simulink library "SCR"  (R2024b)
settings: Solver=VariableStepAuto  StartTime=0.0  StopTime=10.0  RelTol=1e-3
libraries: nesl_utility x29, fl_lib x26, sm_lib x16, ee_lib x7, slpidlib x4
(part 2 of 2)

== system SCR/PID Controller ==
  q1 : Inport
  Q_dorit : Inport  Port=2
  q2 : Inport  Port=3
  Add : Sum  Inputs=-+
  Add1 : Sum  Inputs=+-
  Demux : Demux  Outputs=2
  Mux : Mux  Inputs=2
  Mux1 : Mux  Inputs=2
  PID Controller : slpidlib/PID Controller  Controller=PID  Form=Parallel  TimeDomain=Continuous-time  UseExternalTs=off  SampleTime=-1  IntegratorMethod=Forward Euler  FilterMethod=Forward Euler  ControllerParametersSource=internal  P=17042.9277196606  I=696153.474275857  UseKiTs=off  D=-7.42275649016862  UseExternalDerivativeSource=off  N=2296.03756262702  UseFilter=on  TunerSelectOption=Transfer Function Based (PID Tuner App)  InitialConditionSource=internal  InitialConditionForIntegrator=0  InitialConditionForFilter=0  DifferentiatorICPrevScaledInput=0  ExternalReset=none  TrackingMode=off  Kt=1  LimitOutput=on  SatLimitsSource=internal  UpperSaturationLimit=24  LowerSaturationLimit=-24  LinearizeAsGain=off  AntiWindupMode=clamping  Kb=10  LimitIntegrator=off  UpperIntegratorSaturationLimit=inf  LowerIntegratorSaturationLimit=-inf  POutMin=[]  POutMax=[]  IOutMin=[]  IOutMax=[]  DOutMin=[]  DOutMax=[]  NOutMin=[]  NOutMax=[]  SumOutMin=[]  SumOutMax=[]  SaturationOutMin=[]  SaturationOutMax=[]  PParamMin=[]  PParamMax=[]  IParamMin=[]  IParamMax=[]  DParamMin=[]  DParamMax=[]  NParamMin=[]  NParamMax=[]  KbParamMin=[]  KbParamMax=[]  KtParamMin=[]  KtParamMax=[]  KbOutMin=[]  KbOutMax=[]  KtOutMin=[]  KtOutMax=[]  IntegratorOutMin=[]  IntegratorOutMax=[]  FilterOutMin=[]  FilterOutMax=[]  SumI1OutMin=[]  SumI1OutMax=[]  SumI2OutMin=[]  SumI2OutMax=[]  SumI3OutMin=[]  SumI3OutMax=[]  SumI4OutMin=[]  SumI4OutMax=[]  SumDOutMin=[]  SumDOutMax=[]  DifferentiatorOutMin=[]  DifferentiatorOutMax=[]  FilterDiffOutCoefMin=[]  FilterDiffOutCoefMax=[]  ReciprocalOutMin=[]  ReciprocalOutMax=[]  SumDenOutMin=[]  SumDenOutMax=[]  SumNumOutMin=[]  SumNumOutMax=[]  DivideOutMin=[]  DivideOutMax=[]  UdiffTsProdOutMin=[]  UdiffTsProdOutMax=[]  NTsProdOutMin=[]  NTsProdOutMax=[]  UintegralTsProdOutMin=[]  UintegralTsProdOutMax=[]  UngainTsProdOutMin=[]  UngainTsProdOutMax=[]  ClampingZeroOutDataTypeStr=Inherit: Inherit via back propagation  ClampingZeroOutMin=[]  ClampingZeroOutMax=[]  FilterDenConstantOutDataTypeStr=Inherit: Inherit via back propagation  FilterDenConstantOutMin=[]  FilterDenConstantOutMax=[]  PCopyOutDataTypeStr=Inherit: Inherit via back propagation  PCopyOutMin=[]  PCopyOutMax=[]  NCopyOutDataTypeStr=Inherit: Inherit via back propagation  NCopyOutMin=[]  NCopyOutMax=[]  IntegratorContinuousStateAttributes=''  IntegratorStateMustResolveToSignalObject=off  IntegratorRTWStateStorageClass=Auto  FilterContinuousStateAttributes=''  FilterStateMustResolveToSignalObject=off  FilterRTWStateStorageClass=Auto  ParallelPVariant=InternalParameters  IdealPVariant=Disabled  IVariant=InternalParameters  DVariant=InternalParameters  IntegratorVariant=Continuous  SatVariant=Enabled  AWVariant=ContClampingParallel  PCopyVariant=Disabled  TRVariant=Disabled  FdbkBlocksVariant=Forward  IdealPFdbkVariant=Disabled  SatFdbkVariant=Disabled  DerivativeFilterVariant=ContFilter  NVariant=InternalParameters  NCopyVariant=Disabled  FilterICVariant=InternalICsFilter  IntegratorICVariant=InternalICs  ExternalResetVariant=Disabled  TRSumVariant=Passthrough  SumFdbkVariant=Disabled  SumVariant=Sum_PID  TsampFilterVariant=InternalTs  TsampNgainVariant=Passthrough  TsampIntegralVariant=Disabled_SignalSpec  ExternalSaturationOutDataTypeStr=Inherit: Same as second input  DerivativeSourceVariant=ErrorSignal  PreIntVariant=InternalPreInt
  PID Controller2 : slpidlib/PID Controller  Controller=PID  Form=Parallel  TimeDomain=Continuous-time  UseExternalTs=off  SampleTime=-1  IntegratorMethod=Forward Euler  FilterMethod=Forward Euler  ControllerParametersSource=internal  P=19726.0931917022  I=877163.671153983  UseKiTs=off  D=28.399075244163  UseExternalDerivativeSource=off  N=2735.67202823723  UseFilter=on  TunerSelectOption=Transfer Function Based (PID Tuner App)  InitialConditionSource=internal  InitialConditionForIntegrator=0  InitialConditionForFilter=0  DifferentiatorICPrevScaledInput=0  ExternalReset=none  TrackingMode=off  Kt=1  LimitOutput=on  SatLimitsSource=internal  UpperSaturationLimit=24  LowerSaturationLimit=-24  LinearizeAsGain=off  AntiWindupMode=clamping  Kb=10  LimitIntegrator=off  UpperIntegratorSaturationLimit=inf  LowerIntegratorSaturationLimit=-inf  POutMin=[]  POutMax=[]  IOutMin=[]  IOutMax=[]  DOutMin=[]  DOutMax=[]  NOutMin=[]  NOutMax=[]  SumOutMin=[]  SumOutMax=[]  SaturationOutMin=[]  SaturationOutMax=[]  PParamMin=[]  PParamMax=[]  IParamMin=[]  IParamMax=[]  DParamMin=[]  DParamMax=[]  NParamMin=[]  NParamMax=[]  KbParamMin=[]  KbParamMax=[]  KtParamMin=[]  KtParamMax=[]  KbOutMin=[]  KbOutMax=[]  KtOutMin=[]  KtOutMax=[]  IntegratorOutMin=[]  IntegratorOutMax=[]  FilterOutMin=[]  FilterOutMax=[]  SumI1OutMin=[]  SumI1OutMax=[]  SumI2OutMin=[]  SumI2OutMax=[]  SumI3OutMin=[]  SumI3OutMax=[]  SumI4OutMin=[]  SumI4OutMax=[]  SumDOutMin=[]  SumDOutMax=[]  DifferentiatorOutMin=[]  DifferentiatorOutMax=[]  FilterDiffOutCoefMin=[]  FilterDiffOutCoefMax=[]  ReciprocalOutMin=[]  ReciprocalOutMax=[]  SumDenOutMin=[]  SumDenOutMax=[]  SumNumOutMin=[]  SumNumOutMax=[]  DivideOutMin=[]  DivideOutMax=[]  UdiffTsProdOutMin=[]  UdiffTsProdOutMax=[]  NTsProdOutMin=[]  NTsProdOutMax=[]  UintegralTsProdOutMin=[]  UintegralTsProdOutMax=[]  UngainTsProdOutMin=[]  UngainTsProdOutMax=[]  ClampingZeroOutDataTypeStr=Inherit: Inherit via back propagation  ClampingZeroOutMin=[]  ClampingZeroOutMax=[]  FilterDenConstantOutDataTypeStr=Inherit: Inherit via back propagation  FilterDenConstantOutMin=[]  FilterDenConstantOutMax=[]  PCopyOutDataTypeStr=Inherit: Inherit via back propagation  PCopyOutMin=[]  PCopyOutMax=[]  NCopyOutDataTypeStr=Inherit: Inherit via back propagation  NCopyOutMin=[]  NCopyOutMax=[]  IntegratorContinuousStateAttributes=''  IntegratorStateMustResolveToSignalObject=off  IntegratorRTWStateStorageClass=Auto  FilterContinuousStateAttributes=''  FilterStateMustResolveToSignalObject=off  FilterRTWStateStorageClass=Auto  ParallelPVariant=InternalParameters  IdealPVariant=Disabled  IVariant=InternalParameters  DVariant=InternalParameters  IntegratorVariant=Continuous  SatVariant=Enabled  AWVariant=ContClampingParallel  PCopyVariant=Disabled  TRVariant=Disabled  FdbkBlocksVariant=Forward  IdealPFdbkVariant=Disabled  SatFdbkVariant=Disabled  DerivativeFilterVariant=ContFilter  NVariant=InternalParameters  NCopyVariant=Disabled  FilterICVariant=InternalICsFilter  IntegratorICVariant=InternalICs  ExternalResetVariant=Disabled  TRSumVariant=Passthrough  SumFdbkVariant=Disabled  SumVariant=Sum_PID  TsampFilterVariant=InternalTs  TsampNgainVariant=Passthrough  TsampIntegralVariant=Disabled_SignalSpec  ExternalSaturationOutDataTypeStr=Inherit: Same as second input  DerivativeSourceVariant=ErrorSignal  PreIntVariant=InternalPreInt
  To Workspace : ToWorkspace  VariableName=comanda  SaveFormat=Timeseries  SampleTime=-1
  To Workspace1 : ToWorkspace  VariableName=erori_Q  SaveFormat=Timeseries  SampleTime=-1
  u1 : Outport
  u2 : Outport  Port=2
  wires:
  Demux/2 -> Add1/1
  Demux/1 -> Add/2
  q1/1 -> Add/1
  Add/1 -> Mux1/1, PID Controller/1
  Q_dorit/1 -> Demux/1
  Add1/1 -> PID Controller2/1, Mux1/2
  q2/1 -> Add1/2
  PID Controller/1 -> Mux/1, u1/1  "u1"
  PID Controller2/1 -> Mux/2, u2/1  "u2"
  Mux/1 -> To Workspace/1
  Mux1/1 -> To Workspace1/1

== system SCR/Q_sensed ==
  q1 : Inport
  q2 : Inport  Port=2
  Mux : Mux  Inputs=2
  q_sensor : Outport
  tag scope: q1=global, q2=global, q_sensor=global
  wires:
  q1/1 -> Mux/1, [q1]
  q2/1 -> Mux/2, [q2]
  Mux/1 -> q_sensor/1, [q_sensor]

== system SCR/SCARA_FD_Holist ==
  u : Inport
  Demux : Demux  Outputs=2
  Demux1 : Demux  Outputs=2
  Demux2 : Demux  Outputs=2
  Integrator : Integrator
  Integrator1 : Integrator
  ddq compute : MATLAB Function  TreatAsAtomicUnit=on
  q1 : Outport
  q2 : Outport  Port=2
  dq1 : Outport  Port=3
  dq2 : Outport  Port=4
  ddq1 : Outport  Port=5
  ddq2 : Outport  Port=6
  wires:
  Demux2/2 -> q2/1, ddq compute/2(q2)
  Demux2/1 -> q1/1
  Integrator1/1 -> Demux2/1
  Demux1/2 -> dq2/1, ddq compute/4(dq2)
  Demux1/1 -> dq1/1, ddq compute/3(dq1)
  Demux/2 -> ddq2/1
  Demux/1 -> ddq1/1
  Integrator/1 -> Integrator1/1, Demux1/1
  u/1 -> ddq compute/1(u)
  ddq compute/1(ddq) -> Demux/1, Integrator/1

== system SCR/SCARA_Foward_Dynamics ==
  tau : Inport
  Demux : Demux  Outputs=2
  Demux1 : Demux  Outputs=2
  Demux2 : Demux  Outputs=2
  Integrator : Integrator
  Integrator1 : Integrator
  ddq compute : MATLAB Function  TreatAsAtomicUnit=on
  q1 : Outport
  q2 : Outport  Port=2
  dq1 : Outport  Port=3
  dq2 : Outport  Port=4
  ddq1 : Outport  Port=5
  ddq2 : Outport  Port=6
  wires:
  ddq compute/1(ddq) -> Integrator/1, Demux/1
  tau/1 -> ddq compute/1(tau)
  Integrator/1 -> Demux1/1, Integrator1/1
  Demux/1 -> ddq1/1
  Demux/2 -> ddq2/1
  Demux1/1 -> ddq compute/3(dq1), dq1/1
  Demux1/2 -> ddq compute/4(dq2), dq2/1
  Integrator1/1 -> Demux2/1
  Demux2/1 -> q1/1
  Demux2/2 -> ddq compute/2(q2), q2/1

== system SCR/SCARA_Inverse_Dynamics ==
  q,dq,ddq : Inport
  Demux : Demux  Outputs=2
  Demux1 : Demux  Outputs=5
  Memory : Memory
  To Workspace : ToWorkspace  VariableName=torque  SaveFormat=Timeseries  SampleTime=-1
  tau compute : MATLAB Function  TreatAsAtomicUnit=on
  Torque Joint1 : Outport
  Torque Joint2 : Outport  Port=2
  wires:
  Memory/1 -> Demux1/1
  Demux1/5 -> tau compute/5(ddq2)
  Demux1/4 -> tau compute/4(dq2)
  Demux1/3 -> tau compute/3(q2)
  Demux1/2 -> tau compute/2(ddq1)
  Demux1/1 -> tau compute/1(dq1)
  q,dq,ddq/1 -> Memory/1
  Demux/1 -> Torque Joint1/1
  Demux/2 -> Torque Joint2/1
  tau compute/1(tau) -> To Workspace/1, Demux/1

== system SCR/Scope current, voltage, RPM ==
  Scope : Scope  NumInputPorts=2
  Scope1 : Scope  NumInputPorts=2
  Scope2 : Scope  NumInputPorts=2
  wires:
  [motorCurrent1] -> Scope/1
  [motorCurrent2] -> Scope/2
  [motorVoltage2] -> Scope1/2
  [motorVoltage1] -> Scope1/1
  [motorRPM1] -> Scope2/1
  [motorRPM2] -> Scope2/2

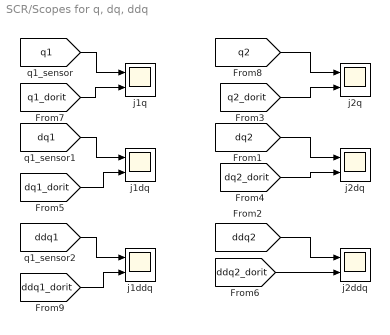
== system SCR/Scopes for q, dq, ddq ==
  j1ddq : Scope  NumInputPorts=2
  j1dq : Scope  NumInputPorts=2
  j1q : Scope  NumInputPorts=2
  j2ddq : Scope  NumInputPorts=2
  j2dq : Scope  NumInputPorts=2
  j2q : Scope  NumInputPorts=2
  wires:
  [dq1] -> j1dq/1
  [q2] -> j2q/1
  [q1] -> j1q/1
  [ddq2] -> j2ddq/1
  [ddq1] -> j1ddq/1
  [dq2] -> j2dq/1
  [dq1_dorit] -> j1dq/2
  [q1_dorit] -> j1q/2
  [ddq1_dorit] -> j1ddq/2
  [q2_dorit] -> j2q/2
  [ddq2_dorit] -> j2ddq/2
  [dq2_dorit] -> j2dq/2

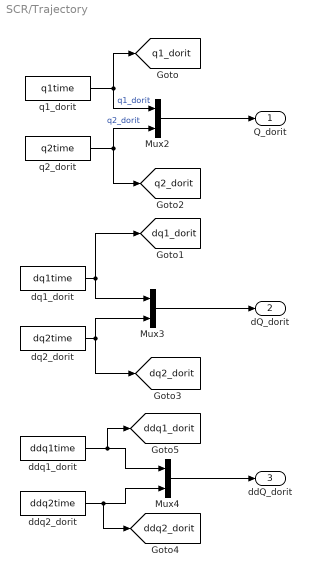
== system SCR/Trajectory ==
  Mux2 : Mux  Inputs=2
  Mux3 : Mux  Inputs=2
  Mux4 : Mux  Inputs=2
  ddq1_dorit : FromWorkspace  VariableName=ddq1time
  ddq2_dorit : FromWorkspace  VariableName=ddq2time
  dq1_dorit : FromWorkspace  VariableName=dq1time
  dq2_dorit : FromWorkspace  VariableName=dq2time
  q1_dorit : FromWorkspace  VariableName=q1time
  q2_dorit : FromWorkspace  VariableName=q2time
  Q_dorit : Outport
  dQ_dorit : Outport  Port=2
  ddQ_dorit : Outport  Port=3
  tag scope: ddq1_dorit=global, ddq2_dorit=global, dq1_dorit=global, dq2_dorit=global, q1_dorit=global, q2_dorit=global
  wires:
  Mux4/1 -> ddQ_dorit/1
  Mux2/1 -> Q_dorit/1
  Mux3/1 -> dQ_dorit/1
  q2_dorit/1 -> Mux2/2, [q2_dorit]  "q2_dorit"
  q1_dorit/1 -> Mux2/1, [q1_dorit]  "q1_dorit"
  dq1_dorit/1 -> [dq1_dorit], Mux3/1
  dq2_dorit/1 -> Mux3/2, [dq2_dorit]
  ddq1_dorit/1 -> [ddq1_dorit], Mux4/1
  ddq2_dorit/1 -> [ddq2_dorit], Mux4/2

== system SCR/actuatorTorques ==
  Actuator Torque 1 : Inport
  Actuator Torque 2 : Inport  Port=2
  Mux : Mux  Inputs=2
  tag scope: actuatorTorque1=global, actuatorTorque2=global, actuatorTorques=global
  wires:
  Actuator Torque 1/1 -> Mux/1, [actuatorTorque1]
  Actuator Torque 2/1 -> Mux/2, [actuatorTorque2]
  Mux/1 -> [actuatorTorques]

== system SCR/dQ_sensed ==
  dq1 : Inport
  dq2 : Inport  Port=2
  Mux1 : Mux  Inputs=2
  dq_sensor : Outport
  tag scope: dq1=global, dq2=global, dq_sensor=global
  wires:
  dq1/1 -> [dq1], Mux1/1
  dq2/1 -> Mux1/2, [dq2]
  Mux1/1 -> dq_sensor/1, [dq_sensor]

== system SCR/ddQ_sensed ==
  ddq1 : Inport
  ddq2 : Inport  Port=2
  Mux1 : Mux  Inputs=2
  tag scope: ddq1=global, ddq2=global, ddq_sensor=global
  wires:
  ddq1/1 -> [ddq1], Mux1/1
  ddq2/1 -> [ddq2], Mux1/2
  Mux1/1 -> [ddq_sensor]

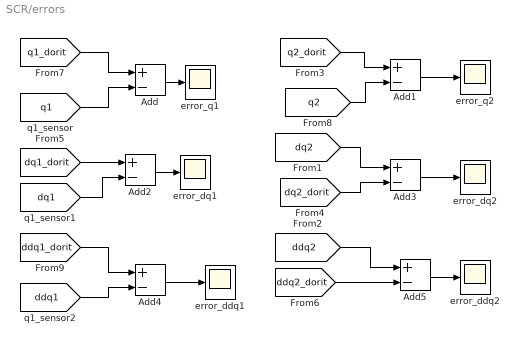
== system SCR/errors ==
  Add{,1..5} (6 alike) : Sum  Inputs=+-
  error_ddq1 : Scope
  error_ddq2 : Scope
  error_dq1 : Scope
  error_dq2 : Scope
  error_q1 : Scope
  error_q2 : Scope
  wires:
  [ddq2] -> Add5/1
  [ddq2_dorit] -> Add5/2
  Add/1 -> error_q1/1
  [q1_dorit] -> Add/1
  [q1] -> Add/2
  [q2_dorit] -> Add1/1
  [q2] -> Add1/2
  Add1/1 -> error_q2/1
  [dq1_dorit] -> Add2/1
  Add2/1 -> error_dq1/1
  [dq1] -> Add2/2
  Add3/1 -> error_dq2/1
  [dq2] -> Add3/1
  [dq2_dorit] -> Add3/2
  [ddq1_dorit] -> Add4/1
  [ddq1] -> Add4/2
  Add4/1 -> error_ddq1/1
  Add5/1 -> error_ddq2/1

== system SCR/Controller_ID/Subsystem ==
  q1 : Inport
  q2 : Inport  Port=2
  dq1 : Inport  Port=3
  dq2 : Inport  Port=4
  MATLAB Function1 : MATLAB Function  TreatAsAtomicUnit=on
  MATLAB Function2 : MATLAB Function  TreatAsAtomicUnit=on
  MATLAB Function3 : MATLAB Function  TreatAsAtomicUnit=on
  M : Outport
  N : Outport  Port=2
  G : Outport  Port=3
  wires:
  MATLAB Function3/1(M) -> M/1
  MATLAB Function1/1(N) -> N/1
  q2/1 -> MATLAB Function2/2(q2), MATLAB Function1/1(q2), MATLAB Function3/1(q2)
  dq2/1 -> MATLAB Function1/3(dq2)
  dq1/1 -> MATLAB Function1/2(dq1)
  MATLAB Function2/1(G) -> G/1
  q1/1 -> MATLAB Function2/1(q1)

== system SCR/Feedfoward/Subsystem ==
  q1 : Inport
  q2 : Inport  Port=2
  dq1 : Inport  Port=3
  dq2 : Inport  Port=4
  MATLAB Function1 : MATLAB Function  TreatAsAtomicUnit=on
  MATLAB Function2 : MATLAB Function  TreatAsAtomicUnit=on
  MATLAB Function3 : MATLAB Function  TreatAsAtomicUnit=on
  M : Outport
  N : Outport  Port=2
  G : Outport  Port=3
  wires:
  MATLAB Function3/1(M) -> M/1
  MATLAB Function1/1(N) -> N/1
  q2/1 -> MATLAB Function2/2(q2), MATLAB Function1/1(q2), MATLAB Function3/1(q2)
  dq2/1 -> MATLAB Function1/3(dq2)
  dq1/1 -> MATLAB Function1/2(dq1)
  MATLAB Function2/1(G) -> G/1
  q1/1 -> MATLAB Function2/1(q1)

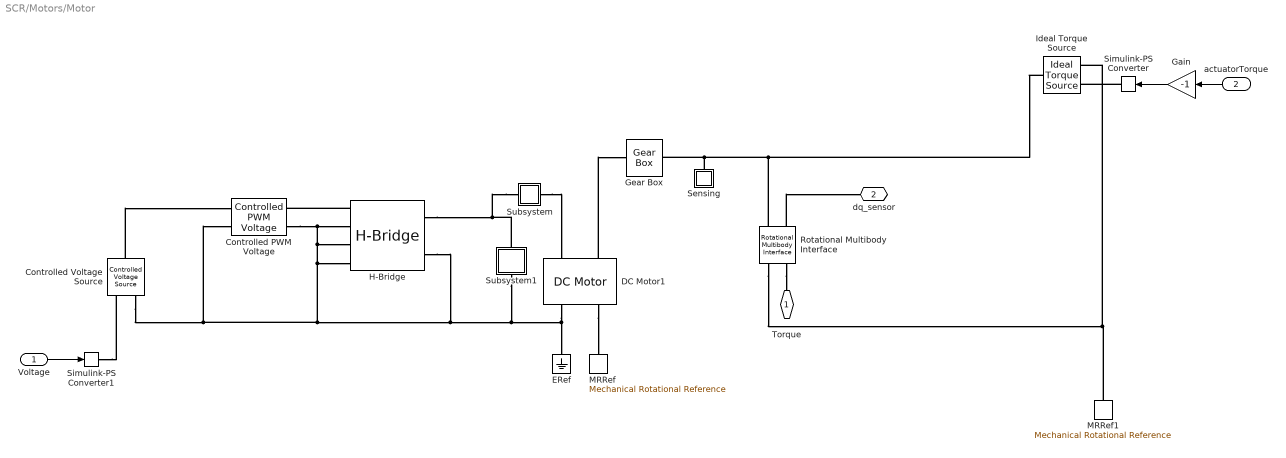
== system SCR/Motors/Motor ==
  Voltage : Inport
  actuatorTorque : Inport  Port=2
  Controlled PWM Voltage : ee_lib/Integrated Circuits/Controlled PWM Voltage  F=4000 Hz  TD=0 s  pulse_width_offset=0 s  pulse_min=0 s  pwm_or_av=ee.enum.pwm_or_av.averaged  event_type=1  sample_time=5e-6 s  Vmin=0 V  Vmax=5 V  Vm=5 V  u_min=0  u_max=1
  Controlled Voltage Source : fl_lib/Electrical/Electrical Sources/Controlled Voltage Source
  DC Motor1 : ee_lib/Electromechanical/Brushed Motors/DC Motor  field_option=ee.enum.field_option.pm  Rf=100 Ohm  Lf=1 H  Laf=0.15 H  If0=0 A  parameterization=ee.enum.dcparam_option.circuit_param  Ra=3.9 Ohm  La=12e-6 H  emf_or_torque=ee.enum.emf_or_torque.kv  Kv=0.072e-3 V/rpm  Ki=6.876e-4 N*m/A  T_stall=0.24e-3 N*m  w_max=19100 rpm  w_rated=15000 rpm  P_rated=0.08 W  V_rated=1.5 V  lam_param=ee.enum.lam_param.damping  i_noload=0 A  V_i_noload=1.5 V  J=0.01 cm^2*g  lam=0 N*m*s/rad  speed0=0 rpm  t_fault_armature=1 s  t_fault_field=1 s  fault_action=simscape.enum.assert.action.none  alpha=3.93e-3 1/K  Tmeas=25 degC  thermal_mass=100 J/K  initial_temperature=25 degC
  ERef : fl_lib/Electrical/Electrical Elements/Electrical Reference
  Gain : Gain  Gain=-1
  Gear Box : fl_lib/Mechanical/Mechanisms/Gear Box  ratio=103  t_in_specify=off  t_in_priority=None  t_in=0 N*m  t_in_nominal_specify=off  t_in_nominal_value=1  t_in_nominal_unit=N*m  t_out_specify=off  t_out_priority=None  t_out=0 N*m  t_out_nominal_specify=off  t_out_nominal_value=1  t_out_nominal_unit=N*m
  H-Bridge : ee_lib/Semiconductors & Converters/Converters/H-Bridge  supply_ports=ee.enum.supply_ports.hidesupply  pwm_or_av=2  regenerative_braking_mode=2  discontinuous=0  freewheeling_mode=1  Rload=3.38+0.1 Ohm  Lload=1e-5 H  F=4 kHz  Venable=2.5 V  Vmax=5 V  Vreverse=2.5 V  Vbrake=2.5 V  Vm=12 V  Ron=0.1 Ohm  Don=0.1 Ohm  Goff=1e-6 S  Tmeas=298.15 K  Ron2=0.1 Ohm  Don2=0.05 Ohm  Tmeas2=398.15 K  thermal_mass=100 J/K  initial_temperature=298.15 K
  Ideal Torque Source : fl_lib/Mechanical/Mechanical Sources/Ideal Torque Source
  MRRef : fl_lib/Mechanical/Rotational Elements/Mechanical Rotational Reference
  MRRef1 : fl_lib/Mechanical/Rotational Elements/Mechanical Rotational Reference
  Rotational Multibody Interface : fl_lib/Mechanical/Multibody Interfaces/Rotational Multibody Interface
  Sensing : Subsystem
      mask Display: disp('w');
  Simulink-PS Converter : nesl_utility/Simulink-PS Converter  PhysicalDomain=network_engine_domain  SubClassName=ps_input  LeftPortType=input  RightPortType=output  PseudoPeriodic=off  Frequencies=[]  NoiseDistribution=none  NoiseParameters=[]  Unit=1  AffineConversion=off  FilteringAndDerivatives=provide  SimscapeFilterOrder=1  InputFilterTimeConstant=0.001  UdotUserProvided=0
  Simulink-PS Converter1 : nesl_utility/Simulink-PS Converter  PhysicalDomain=network_engine_domain  SubClassName=ps_input  LeftPortType=input  RightPortType=output  PseudoPeriodic=off  Frequencies=[]  NoiseDistribution=none  NoiseParameters=[]  Unit=1  AffineConversion=off  FilteringAndDerivatives=provide  SimscapeFilterOrder=1  InputFilterTimeConstant=0.001  UdotUserProvided=0
  Subsystem : Subsystem
      mask Display: disp("A")
  Subsystem1 : Subsystem
      mask Display: disp("V")
  Torque : PMIOPort  Side=Left
  dq_sensor : PMIOPort  Port=2  Side=Right
  wires:
  Voltage/1 -> Simulink-PS Converter1/1
  Gain/1 -> Simulink-PS Converter/1
  actuatorTorque/1 -> Gain/1
  connections:
  Subsystem/RConn1 -- DC Motor1/LConn1
  Simulink-PS Converter1/RConn1 -- Controlled Voltage Source/RConn1
  Simulink-PS Converter/RConn1 -- Ideal Torque Source/RConn1
  Ideal Torque Source/RConn2 -- MRRef1/LConn1 -- Rotational Multibody Interface/LConn2
  Rotational Multibody Interface/LConn1 -- Torque/RConn1
  Rotational Multibody Interface/RConn1 -- dq_sensor/RConn1
  Controlled Voltage Source/LConn1 -- Controlled PWM Voltage/LConn1
  Subsystem/LConn1 -- Subsystem1/LConn1 -- H-Bridge/RConn1
  Subsystem1/RConn1 -- H-Bridge/RConn2 -- Controlled PWM Voltage/RConn2 -- H-Bridge/LConn2 -- H-Bridge/LConn3 -- H-Bridge/LConn4 -- Controlled PWM Voltage/LConn2 -- Controlled Voltage Source/RConn2 -- DC Motor1/RConn1 -- ERef/LConn1
  Ideal Torque Source/LConn1 -- Rotational Multibody Interface/RConn2 -- Sensing/LConn1 -- Gear Box/RConn1
  DC Motor1/RConn2 -- MRRef/LConn1
  H-Bridge/LConn1 -- Controlled PWM Voltage/RConn1
  DC Motor1/LConn2 -- Gear Box/LConn1

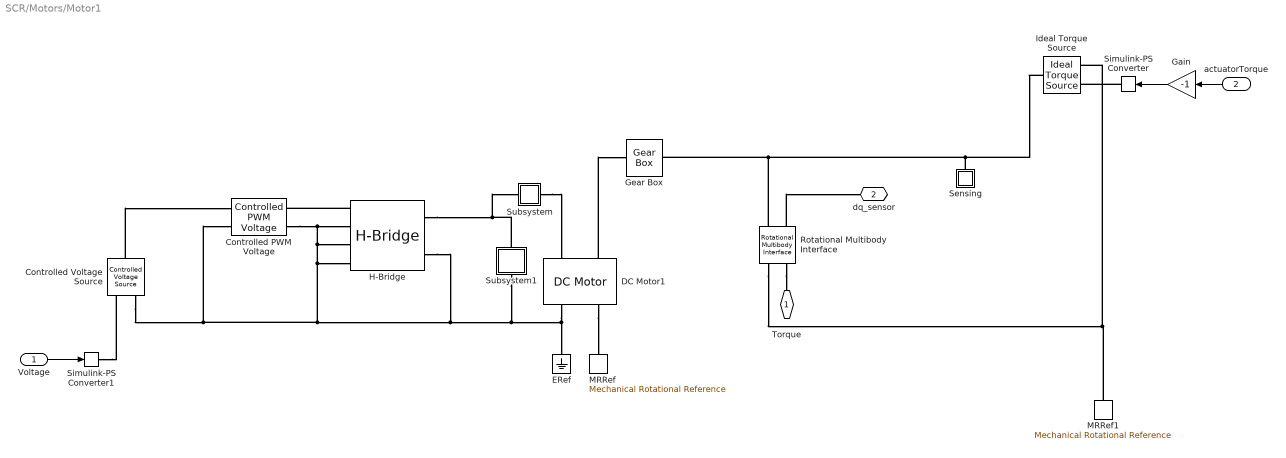
== system SCR/Motors/Motor1 ==
  Voltage : Inport
  actuatorTorque : Inport  Port=2
  Controlled PWM Voltage : ee_lib/Integrated Circuits/Controlled PWM Voltage  F=4000 Hz  TD=0 s  pulse_width_offset=0 s  pulse_min=0 s  pwm_or_av=ee.enum.pwm_or_av.averaged  event_type=1  sample_time=5e-6 s  Vmin=0 V  Vmax=5 V  Vm=5 V  u_min=0  u_max=1
  Controlled Voltage Source : fl_lib/Electrical/Electrical Sources/Controlled Voltage Source
  DC Motor1 : ee_lib/Electromechanical/Brushed Motors/DC Motor  field_option=ee.enum.field_option.pm  Rf=100 Ohm  Lf=1 H  Laf=0.15 H  If0=0 A  parameterization=ee.enum.dcparam_option.circuit_param  Ra=3.9 Ohm  La=12e-6 H  emf_or_torque=ee.enum.emf_or_torque.kv  Kv=0.072e-3 V/rpm  Ki=6.876e-4 N*m/A  T_stall=0.24e-3 N*m  w_max=19100 rpm  w_rated=15000 rpm  P_rated=0.08 W  V_rated=1.5 V  lam_param=ee.enum.lam_param.damping  i_noload=0 A  V_i_noload=1.5 V  J=0.01 cm^2*g  lam=0 N*m*s/rad  speed0=0 rpm  t_fault_armature=1 s  t_fault_field=1 s  fault_action=simscape.enum.assert.action.none  alpha=3.93e-3 1/K  Tmeas=25 degC  thermal_mass=100 J/K  initial_temperature=25 degC
  ERef : fl_lib/Electrical/Electrical Elements/Electrical Reference
  Gain : Gain  Gain=-1
  Gear Box : fl_lib/Mechanical/Mechanisms/Gear Box  ratio=103  t_in_specify=off  t_in_priority=None  t_in=0 N*m  t_in_nominal_specify=off  t_in_nominal_value=1  t_in_nominal_unit=N*m  t_out_specify=off  t_out_priority=None  t_out=0 N*m  t_out_nominal_specify=off  t_out_nominal_value=1  t_out_nominal_unit=N*m
  H-Bridge : ee_lib/Semiconductors & Converters/Converters/H-Bridge  supply_ports=ee.enum.supply_ports.hidesupply  pwm_or_av=2  regenerative_braking_mode=2  discontinuous=0  freewheeling_mode=1  Rload=3.38+0.1 Ohm  Lload=1e-5 H  F=4 kHz  Venable=2.5 V  Vmax=5 V  Vreverse=2.5 V  Vbrake=2.5 V  Vm=12 V  Ron=0.1 Ohm  Don=0.1 Ohm  Goff=1e-6 S  Tmeas=298.15 K  Ron2=0.1 Ohm  Don2=0.05 Ohm  Tmeas2=398.15 K  thermal_mass=100 J/K  initial_temperature=298.15 K
  Ideal Torque Source : fl_lib/Mechanical/Mechanical Sources/Ideal Torque Source
  MRRef : fl_lib/Mechanical/Rotational Elements/Mechanical Rotational Reference
  MRRef1 : fl_lib/Mechanical/Rotational Elements/Mechanical Rotational Reference
  Rotational Multibody Interface : fl_lib/Mechanical/Multibody Interfaces/Rotational Multibody Interface
  Sensing : Subsystem
      mask Display: disp('w');
  Simulink-PS Converter : nesl_utility/Simulink-PS Converter  PhysicalDomain=network_engine_domain  SubClassName=ps_input  LeftPortType=input  RightPortType=output  PseudoPeriodic=off  Frequencies=[]  NoiseDistribution=none  NoiseParameters=[]  Unit=1  AffineConversion=off  FilteringAndDerivatives=provide  SimscapeFilterOrder=1  InputFilterTimeConstant=0.001  UdotUserProvided=0
  Simulink-PS Converter1 : nesl_utility/Simulink-PS Converter  PhysicalDomain=network_engine_domain  SubClassName=ps_input  LeftPortType=input  RightPortType=output  PseudoPeriodic=off  Frequencies=[]  NoiseDistribution=none  NoiseParameters=[]  Unit=1  AffineConversion=off  FilteringAndDerivatives=provide  SimscapeFilterOrder=1  InputFilterTimeConstant=0.001  UdotUserProvided=0
  Subsystem : Subsystem
      mask Display: disp("A")
  Subsystem1 : Subsystem
      mask Display: disp("V")
  Torque : PMIOPort  Side=Left
  dq_sensor : PMIOPort  Port=2  Side=Right
  wires:
  Voltage/1 -> Simulink-PS Converter1/1
  Gain/1 -> Simulink-PS Converter/1
  actuatorTorque/1 -> Gain/1
  connections:
  Subsystem/RConn1 -- DC Motor1/LConn1
  Simulink-PS Converter1/RConn1 -- Controlled Voltage Source/RConn1
  Simulink-PS Converter/RConn1 -- Ideal Torque Source/RConn1
  Ideal Torque Source/RConn2 -- MRRef1/LConn1 -- Rotational Multibody Interface/LConn2
  Rotational Multibody Interface/LConn1 -- Torque/RConn1
  Rotational Multibody Interface/RConn1 -- dq_sensor/RConn1
  Controlled Voltage Source/LConn1 -- Controlled PWM Voltage/LConn1
  Subsystem1/LConn1 -- Subsystem/LConn1 -- H-Bridge/RConn1
  DC Motor1/RConn1 -- Subsystem1/RConn1 -- H-Bridge/RConn2 -- Controlled PWM Voltage/RConn2 -- H-Bridge/LConn2 -- H-Bridge/LConn3 -- H-Bridge/LConn4 -- Controlled PWM Voltage/LConn2 -- Controlled Voltage Source/RConn2 -- ERef/LConn1
  Gear Box/RConn1 -- Rotational Multibody Interface/RConn2 -- Sensing/LConn1 -- Ideal Torque Source/LConn1
  DC Motor1/RConn2 -- MRRef/LConn1
  H-Bridge/LConn1 -- Controlled PWM Voltage/RConn1
  DC Motor1/LConn2 -- Gear Box/LConn1

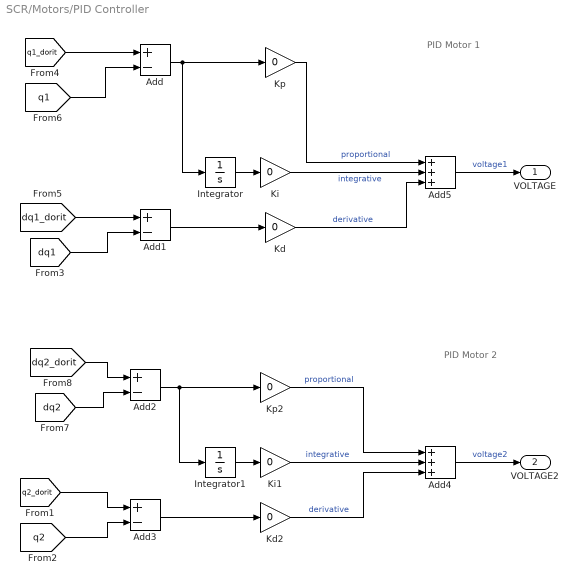
== system SCR/Motors/PID Controller ==
  note: PID Motor 1
  note: PID Motor 2
  Add{,1..3} (4 alike) : Sum  Inputs=+-
  Add4 : Sum  Inputs=+++
  Add5 : Sum  Inputs=+++
  Integrator : Integrator
  Integrator1 : Integrator
  Kd : Gain  Gain=0
  Kd2 : Gain  Gain=0
  Ki : Gain  Gain=0
  Ki1 : Gain  Gain=0
  Kp : Gain  Gain=0
  Kp2 : Gain  Gain=0
  VOLTAGE : Outport
  VOLTAGE2 : Outport  Port=2
  wires:
  Add1/1 -> Kd/1
  [q1] -> Add/2
  [dq1] -> Add1/2
  [q1_dorit] -> Add/1
  Kd/1 -> Add5/3  "derivative"
  [dq1_dorit] -> Add1/1
  Add5/1 -> VOLTAGE/1  "voltage1"
  Kp/1 -> Add5/1  "proportional"
  Ki/1 -> Add5/2  "integrative"
  Add/1 -> Kp/1, Integrator/1
  Integrator/1 -> Ki/1
  Kp2/1 -> Add4/1  "proportional"
  Ki1/1 -> Add4/2  "integrative"
  Integrator1/1 -> Ki1/1
  [dq2_dorit] -> Add2/1
  Add4/1 -> VOLTAGE2/1  "voltage2"
  [q2] -> Add3/2
  Add3/1 -> Kd2/1
  Kd2/1 -> Add4/3  "derivative"
  [dq2] -> Add2/2
  [q2_dorit] -> Add3/1
  Add2/1 -> Integrator1/1, Kp2/1

== system SCR/Motors/Motor/Sensing ==
  Ideal Rotational Motion Sensor : fl_lib/Mechanical/Mechanical Sensors/Ideal Rotational Motion Sensor  reference=foundation.enum.MeasurementReference.difference  acceleration_port=false  velocity_port=true  position_port=true  wrap_angle=simscape.enum.onoff.off  offset=0 rad
  Mechanical Rotational Reference2 : fl_lib/Mechanical/Rotational Elements/Mechanical Rotational Reference
  PS-Simulink Converter 1 : nesl_utility/PS-Simulink Converter  PhysicalDomain=network_engine_domain  SubClassName=ps_output  LeftPortType=input  RightPortType=output  PseudoPeriodic=off  Frequencies=[]  VectorFormat=1-D array  Unit=rpm  AffineConversion=off
  R : PMIOPort  Side=Left
  tag scope: motorRPM1=global
  wires:
  PS-Simulink Converter 1/1 -> [motorRPM1]
  connections:
  R/RConn1 -- Ideal Rotational Motion Sensor/LConn1
  Mechanical Rotational Reference2/LConn1 -- Ideal Rotational Motion Sensor/RConn1
  Ideal Rotational Motion Sensor/RConn2 -- PS-Simulink Converter 1/LConn1

== system SCR/Motors/Motor/Subsystem ==
  Current Sensor1 : fl_lib/Electrical/Electrical Sensors/Current Sensor
  PS-Simulink Converter2 : nesl_utility/PS-Simulink Converter  PhysicalDomain=network_engine_domain  SubClassName=ps_output  LeftPortType=input  RightPortType=output  PseudoPeriodic=off  Frequencies=[]  VectorFormat=inherit  Unit=inherit  AffineConversion=off
  Conn1 : PMIOPort  Side=Left
  Conn2 : PMIOPort  Port=2  Side=Right
  tag scope: motorCurrent1=global
  wires:
  PS-Simulink Converter2/1 -> [motorCurrent1]
  connections:
  Conn1/RConn1 -- Current Sensor1/LConn1
  Current Sensor1/RConn2 -- Conn2/RConn1
  PS-Simulink Converter2/LConn1 -- Current Sensor1/RConn1

== system SCR/Motors/Motor/Subsystem1 ==
  PS-Simulink Converter1 : nesl_utility/PS-Simulink Converter  PhysicalDomain=network_engine_domain  SubClassName=ps_output  LeftPortType=input  RightPortType=output  PseudoPeriodic=off  Frequencies=[]  VectorFormat=inherit  Unit=inherit  AffineConversion=off
  Voltage Sensor : fl_lib/Electrical/Electrical Sensors/Voltage Sensor
  Conn1 : PMIOPort  Side=Left
  Conn2 : PMIOPort  Port=2  Side=Right
  tag scope: motorVoltage1=global
  wires:
  PS-Simulink Converter1/1 -> [motorVoltage1]
  connections:
  Voltage Sensor/RConn2 -- Conn2/RConn1
  PS-Simulink Converter1/LConn1 -- Voltage Sensor/RConn1
  Voltage Sensor/LConn1 -- Conn1/RConn1

== system SCR/Motors/Motor1/Sensing ==
  Ideal Rotational Motion Sensor : fl_lib/Mechanical/Mechanical Sensors/Ideal Rotational Motion Sensor  reference=foundation.enum.MeasurementReference.difference  acceleration_port=false  velocity_port=true  position_port=true  wrap_angle=simscape.enum.onoff.off  offset=0 rad
  Mechanical Rotational Reference2 : fl_lib/Mechanical/Rotational Elements/Mechanical Rotational Reference
  PS-Simulink Converter 1 : nesl_utility/PS-Simulink Converter  PhysicalDomain=network_engine_domain  SubClassName=ps_output  LeftPortType=input  RightPortType=output  PseudoPeriodic=off  Frequencies=[]  VectorFormat=1-D array  Unit=rpm  AffineConversion=off
  R : PMIOPort  Side=Left
  tag scope: motorRPM2=global
  wires:
  PS-Simulink Converter 1/1 -> [motorRPM2]
  connections:
  R/RConn1 -- Ideal Rotational Motion Sensor/LConn1
  Mechanical Rotational Reference2/LConn1 -- Ideal Rotational Motion Sensor/RConn1
  Ideal Rotational Motion Sensor/RConn2 -- PS-Simulink Converter 1/LConn1

== system SCR/Motors/Motor1/Subsystem ==
  Current Sensor1 : fl_lib/Electrical/Electrical Sensors/Current Sensor
  PS-Simulink Converter2 : nesl_utility/PS-Simulink Converter  PhysicalDomain=network_engine_domain  SubClassName=ps_output  LeftPortType=input  RightPortType=output  PseudoPeriodic=off  Frequencies=[]  VectorFormat=inherit  Unit=inherit  AffineConversion=off
  Conn1 : PMIOPort  Side=Left
  Conn2 : PMIOPort  Port=2  Side=Right
  tag scope: motorCurrent2=global
  wires:
  PS-Simulink Converter2/1 -> [motorCurrent2]
  connections:
  Conn1/RConn1 -- Current Sensor1/LConn1
  Current Sensor1/RConn2 -- Conn2/RConn1
  PS-Simulink Converter2/LConn1 -- Current Sensor1/RConn1

== system SCR/Motors/Motor1/Subsystem1 ==
  PS-Simulink Converter1 : nesl_utility/PS-Simulink Converter  PhysicalDomain=network_engine_domain  SubClassName=ps_output  LeftPortType=input  RightPortType=output  PseudoPeriodic=off  Frequencies=[]  VectorFormat=inherit  Unit=inherit  AffineConversion=off
  Voltage Sensor : fl_lib/Electrical/Electrical Sensors/Voltage Sensor
  Conn1 : PMIOPort  Side=Left
  Conn2 : PMIOPort  Port=2  Side=Right
  tag scope: motorVoltage2=global
  wires:
  PS-Simulink Converter1/1 -> [motorVoltage2]
  connections:
  Voltage Sensor/RConn2 -- Conn2/RConn1
  PS-Simulink Converter1/LConn1 -- Voltage Sensor/RConn1
  Voltage Sensor/LConn1 -- Conn1/RConn1

== matlab function SCR/Motor1/MATLAB Function ==
  data: tau input; ddq output; u input; dq input
function ddq = Motor(tau, u, dq)
    b = 0.1; %[Nms/rad]
    k_M = 27.3*10^-3; %[mNm/A]
    randament = 1/1.74; 
    i_r = 103;
    R = 0.200; %[ohm]
    J_a = 72.8*10^-6; %[gcm^2]


    factor1 = (b + k_M^2/R)*dq;
    factor2 = tau/(randament*i_r^2);
    factor3 = k_M / (i_r * R) * u;
    ddq = 1/J_a * (factor3 - factor1 - factor2);

== matlab function SCR/Motor2/MATLAB Function1 ==
  data: tau input; ddq output; u input; dq input
function ddq = Motor(tau, u, dq)
    b = 0.1; %[Nms/rad]
    k_M = 27.3*10^-3; %[mNm/A]
    randament = 1/1.74; 
    i_r = 103;
    R = 0.200; %[ohm]
    J_a = 72.8*10^-6; %[gcm^2]


    factor1 = (b + k_M^2/R)*dq;
    factor2 = tau/(randament*i_r^2);
    factor3 = k_M / (i_r * R) * u;
    ddq = 1/J_a * (factor3 - factor1 - factor2);

== matlab function SCR/Controller_ID_Holist/MATLAB Function ==
  data: u output; q2 input; dq1 input; dq2 input; e input; ddQ_dorit input
function u = controlul_DI(q2, dq1, dq2, e, ddQ_dorit)
    % parametri structura
    m1 = 1;      
    m2 = 2;      
    l1 = 0.2;
    lc2 = 0.1;
    lc1 = 0.1;
    Izz1 = 3.68e-3;
    Izz2 = 7.366e-3;

    % parametri motor
    J_t = 72.8e-6;
    i_r = 103;
    n = 1/1.74;
    b = 0.1;
    k_M = 27.3e-3;
    R = 0.108;

    factor1 = diag(1/(n*i_r^2));
    factor2 = diag(b + k_M^2/R);
    factor3 = diag(k_M/(i_r*R));
    factor4 = inv(diag(k_M/(i_r*R)));
    

    M = factor4  * (diag(J_t) + factor1 * [m2*l1^2 + 2*m2*cos(q2)*l1*lc2 + m1*lc1^2 + m2*lc2^2 + Izz1 + Izz2, m2*lc2^2 + l1*m2*cos(q2)*lc2 + Izz2; 
     m2*lc2^2 + l1*m2*cos(q2)*lc2 + Izz2, m2*lc2^2 + Izz2]);


    % coriolis
    B_coriolis = [-2*l1*lc2*m2*sin(q2);
         0];

    
    % centrifugal
    Cn = [0, -l1*lc2*m2*sin(q2);
          l1*lc2*m2*sin(q2), 0];


    N = Cn*[dq1^2; dq2^2] + B_coriolis*dq1*dq2;
    N = factor4 * factor1 * N;

    B = factor4 * factor2;
    B = B * [dq1; dq2];
    


    % gravitational
    G = [0;0];

    u = M*(e+ddQ_dorit) + B + N;

== matlab function SCR/SCARA_FD_Holist/ddq compute ==
  data: u input; ddq output; q2 input; dq1 input; dq2 input
function ddq = foward_dynamics(u, q2, dq1, dq2)
    % parametri structura
    m1 = 1;      
    m2 = 2;      
    l1 = 0.2;
    lc2 = 0.1;
    lc1 = 0.1;
    Izz1 = 3.68e-3;
    Izz2 = 7.366e-3;
    
    % parametri motor
    J_t = 72.8e-6;
    i_r = 103;
    n = 1/1.74;
    b = 0.1;
    k_M = 27.3e-3;
    R = 0.108;


    factor1 = diag(1/(n*i_r^2));
    factor2 = diag(b + k_M^2/R);
    factor3 = diag(1/(n*i_r^2));
    factor4 = diag(k_M/(i_r*R));

    % mass inertia
    M = diag(J_t) +  factor1 * [m2*l1^2 + 2*m2*cos(q2)*l1*lc2 + m1*lc1^2 + m2*lc2^2 + Izz1 + Izz2, m2*lc2^2 + l1*m2*cos(q2)*lc2 + Izz2; 
     m2*lc2^2 + l1*m2*cos(q2)*lc2 + Izz2, m2*lc2^2 + Izz2];

     % coriolis
    B_coriolis = [-2*l1*lc2*m2*sin(q2);
         0];
    
    % centrifugal
    Cn = [0, -l1*lc2*m2*sin(q2);
          l1*lc2*m2*sin(q2), 0];
    % coriolis + centrifugal
    N = Cn*[dq1^2; dq2^2] + B_coriolis*dq1*dq2;

    N = factor3 * N;
    
    % comanda
    u = factor4 * u;

    B = factor2 * [dq1; dq2];
    
    % gravitationalul
    G = [0;0];

    ddq = inv(M) * (u - N - B - G);

== matlab function SCR/Feedfoward/Subsystem/MATLAB Function1 ==
  data: N output; q2 input; dq1 input; dq2 input
function N = velocityProductTorque(q2, dq1, dq2)
 
    m2 = 1.6;      
    l1 = 0.18;
    lc2 = 0.09;


    % coriolis
    B = [-2*l1*lc2*m2*sin(q2);
         0];
    velocity_vector = dq1*dq2;
    
    % centrifugal
    Cn = [0, -l1*lc2*m2*sin(q2);
          l1*lc2*m2*sin(q2), 0];
    velocity_vector_squared = [dq1^2; dq2^2];
    

    N = Cn*velocity_vector_squared + B*velocity_vector;
end

== matlab function SCR/Feedfoward/Subsystem/MATLAB Function2 ==
  data: q1 input; G output; q2 input
function G = gravity(q1, q2)

    
    m1 = 1.6;      
    m2 = 1.6;        
    l1 = 0.18;
    lc1 = 0.09;
    lc2 = 0.09;
    g = 9.82;
    
    G = [0;0];

end

== matlab function SCR/Controller_ID/Subsystem/MATLAB Function1 ==
  data: N output; q2 input; dq1 input; dq2 input
function N = velocityProductTorque(q2, dq1, dq2)
 
    m2 = 1.6;      
    l1 = 0.18;
    lc2 = 0.09;

    % coriolis
    B = [-2*l1*lc2*m2*sin(q2);
         0];
    
    % centrifugal
    Cn = [0, -l1*lc2*m2*sin(q2);
          l1*lc2*m2*sin(q2), 0]; 

    N = Cn*[dq1^2; dq2^2]; + B*[dq1*dq2];
end

== matlab function SCR/Controller_ID/Subsystem/MATLAB Function2 ==
  data: q1 input; G output; q2 input
function G = gravity(q1, q2)

    
    m1 = 1.6;      
    m2 = 1.6;        
    l1 = 0.18;
    lc1 = 0.09;
    lc2 = 0.09;
    g = 9.82;
    
    G = [0;0];

end

== matlab function SCR/Controller_ID/Subsystem/MATLAB Function3 ==
  data: q2 input; M output
function M = massInertia(q2)

    m1 = 1.6;      
    m2 = 1.6;      
    l1 = 0.18;
    lc2 = 0.09;
    lc1 = 0.09;
    Izz1 = 0.05;
    Izz2 = 0.05;

    M = [m2*l1^2 + 2*m2*cos(q2)*l1*lc2 + m1*lc1^2 + m2*lc2^2 + Izz1 + Izz2, m2*lc2^2 + l1*m2*cos(q2)*lc2 + Izz2; 
     m2*lc2^2 + l1*m2*cos(q2)*lc2 + Izz2, m2*lc2^2 + Izz2];
end

== matlab function SCR/Feedfoward/Subsystem/MATLAB Function3 ==
  data: q2 input; M output
function M = massInertia(q2)

    m1 = 1.6;      
    m2 = 1.6;      
    l1 = 0.18;
    lc2 = 0.09;
    lc1 = 0.09;
    Izz1 = 0.05;
    Izz2 = 0.05;

    M = [m2*l1^2 + 2*m2*cos(q2)*l1*lc2 + m1*lc1^2 + m2*lc2^2 + Izz1 + Izz2, m2*lc2^2 + l1*m2*cos(q2)*lc2 + Izz2; 
     m2*lc2^2 + l1*m2*cos(q2)*lc2 + Izz2, m2*lc2^2 + Izz2];
end

== matlab function SCR/Motors Mathematical Model/MATLAB Function ==
  data: tau input; ddq output; u input; dq input
function ddq = Motor(tau, u, dq)
    b = 0.1; %[Nms/rad]
    k_M = 27.3 * 10^-3; %[mNm/A]
    randament = 1/1.74; 
    i_r = 103;
    R = 0.331; %[ohm]
    J_a = 72.8 * 10^-6; %[gcm^2]


    factor1 = (b + k_M^2/R)*dq;
    factor2 = tau/(randament*i_r^2);
    factor3 = k_M / (i_r * R) * u;
    ddq = 1/J_a * (factor3 - factor1 - factor2);

== matlab function SCR/Motors Mathematical Model/MATLAB Function1 ==
  data: tau input; ddq output; u input; dq input
function ddq = Motor(tau, u, dq)
    b = 0.1; %[Nms/rad]
    k_M = 27.3; %[mNm/A]
    randament = 1/1.74; 
    i_r = 103;
    R = 0.331; %[ohm]
    J_a = 72.8; %[gcm^2]


    factor1 = (b + k_M^2/R)*dq;
    factor2 = tau/(randament*i_r^2);
    factor3 = k_M / (i_r * R) * u;
    ddq = 1/J_a * (factor3 - factor1 - factor2);

== matlab function SCR/SCARA_Inverse_Dynamics/tau compute ==
  data: dq1 input; ddq1 input; q2 input; tau output; dq2 input; ddq2 input
function tau = tau_compute(dq1, ddq1, q2, dq2, ddq2)
    
    % parametri structura
    m1 = 1;      
    m2 = 2;      
    l1 = 0.2;
    lc2 = 0.1;
    lc1 = 0.1;
    Izz1 = 3.68e-3;
    Izz2 = 7.366e-3;
   
    % mass inertia
    M = [m2*l1^2 + 2*m2*cos(q2)*l1*lc2 + m1*lc1^2 + m2*lc2^2 + Izz1 + Izz2, m2*lc2^2 + l1*m2*cos(q2)*lc2 + Izz2; 
     m2*lc2^2 + l1*m2*cos(q2)*lc2 + Izz2, m2*lc2^2 + Izz2];
    M = M * [ddq1; ddq2];

     % coriolis
    B_coriolis = [-2*l1*lc2*m2*sin(q2);
         0];
    
    % centrifugal
    Cn = [0, -l1*lc2*m2*sin(q2);
          l1*lc2*m2*sin(q2), 0];
    % coriolis + centrifugal
    N = Cn*[dq1^2; dq2^2] + B_coriolis*dq1*dq2;

    G = [0;0];

    tau = M + N + G;

== matlab function SCR/SCARA_Foward_Dynamics/ddq compute ==
  data: tau input; ddq output; q2 input; dq1 input; dq2 input
function ddq = foward_dynamics(tau, q2, dq1, dq2)
    m1 = 1;      
    m2 = 2;      
    l1 = 0.2;
    lc2 = 0.1;
    lc1 = 0.1;
    Izz1 = 3.68e-3;
    Izz2 = 7.366e-3;

    % mass inertia
    M = [m2*l1^2 + 2*m2*cos(q2)*l1*lc2 + m1*lc1^2 + m2*lc2^2 + Izz1 + Izz2, m2*lc2^2 + l1*m2*cos(q2)*lc2 + Izz2; 
     m2*lc2^2 + l1*m2*cos(q2)*lc2 + Izz2, m2*lc2^2 + Izz2];

     % coriolis
    B = [-2*l1*lc2*m2*sin(q2);
         0];
    
    % centrifugal
    Cn = [0, -l1*lc2*m2*sin(q2);
          l1*lc2*m2*sin(q2), 0];

    N = Cn*[dq1^2; dq2^2] + B*dq1*dq2;

    G = [0;0];

    ddq = inv(M) * (tau - N - G);
